simulink model "AC_DCj_iaocuo_simple_hysteresis_1V_commutation_softstart_tuned"  (R2024b)
settings: Solver=FixedStepDiscrete  StartTime=0.0  StopTime=1  FixedStep=1e-7  RelTol=1e-3
libraries: spsMosfetLib x6, spsCurrentMeasurementLib x4, spsSeriesRLCBranchLib x4, slpidlib x3, simulink x3, spsVoltageMeasurementLib x2, spsACVoltageSourceLib x1, dspstat3 x1, sps_lib x1
settings Model: Creator=YuJian  LastModifiedBy=YuJian
settings DataIOCC: ReturnWorkspaceOutputs=off

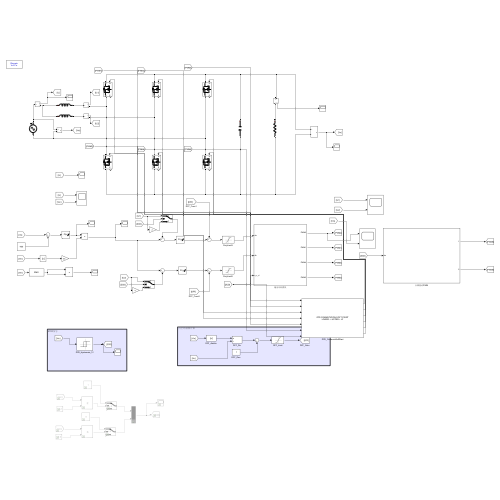
[thumbnail: Simulink's stored preview of the top-level diagram]
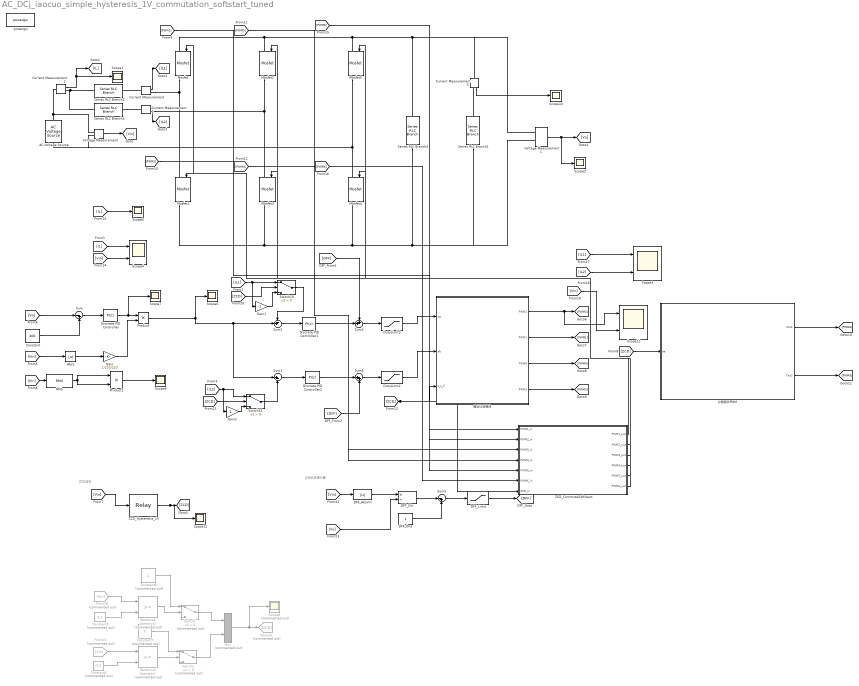
== system AC_DCj_iaocuo_simple_hysteresis_1V_commutation_softstart_tuned ==
  note: 占空比前馈计算
  note: ZCD信号
  AC Voltage Source : spsACVoltageSourceLib/AC Voltage Source  Amplitude=311  Phase=0  Frequency=50  SampleTime=0  Measurements=None  BusType=swing  Pref=10e3  Qref=0  Qmin=-inf  Qmax=+inf
  Abs1 : Abs  SaturateOnIntegerOverflow=off
  Constant : Constant  Value=400
  Constant2 : Constant  Commented=on  Value=-0.2
  Constant5 : Constant  Commented=on  Value=0.2
  Constant6 : Constant  Commented=on
  Constant7 : Constant  Commented=on  Value=0
  Current Measurement{,1..3} (4 alike) : spsCurrentMeasurementLib/Current Measurement  PhasorSimulation=off  OutputType=Complex  PSBequivalent=0
  DFF_AbsVin : Abs  SaturateOnIntegerOverflow=off
  DFF_Div : Product  Inputs=*/
  DFF_Limit : Saturate  UpperLimit=1  LowerLimit=0
  DFF_One : Constant
  Discrete PID Controller : slpidlib/PID Controller  Controller=PI  Form=Parallel  TimeDomain=Discrete-time  UseExternalTs=off  SampleTime=-1  IntegratorMethod=Forward Euler  FilterMethod=Forward Euler  ControllerParametersSource=internal  P=4  I=230  UseKiTs=off  D=0  UseExternalDerivativeSource=off  N=100  UseFilter=on  TunerSelectOption=Transfer Function Based (PID Tuner App)  InitialConditionSource=internal  InitialConditionForIntegrator=0  InitialConditionForFilter=0  DifferentiatorICPrevScaledInput=0  ExternalReset=none  TrackingMode=off  Kt=1  LimitOutput=on  SatLimitsSource=internal  UpperSaturationLimit=5500  LowerSaturationLimit=0  LinearizeAsGain=off  AntiWindupMode=clamping  Kb=1  LimitIntegrator=off  UpperIntegratorSaturationLimit=inf  LowerIntegratorSaturationLimit=-inf  POutMin=[]  POutMax=[]  IOutMin=[]  IOutMax=[]  DOutMin=[]  DOutMax=[]  NOutMin=[]  NOutMax=[]  SumOutMin=[]  SumOutMax=[]  SaturationOutMin=[]  SaturationOutMax=[]  PParamMin=[]  PParamMax=[]  IParamMin=[]  IParamMax=[]  DParamMin=[]  DParamMax=[]  NParamMin=[]  NParamMax=[]  KbParamMin=[]  KbParamMax=[]  KtParamMin=[]  KtParamMax=[]  KbOutMin=[]  KbOutMax=[]  KtOutMin=[]  KtOutMax=[]  IntegratorOutMin=[]  IntegratorOutMax=[]  FilterOutMin=[]  FilterOutMax=[]  SumI1OutMin=[]  SumI1OutMax=[]  SumI2OutMin=[]  SumI2OutMax=[]  SumI3OutMin=[]  SumI3OutMax=[]  SumI4OutMin=[]  SumI4OutMax=[]  SumDOutMin=[]  SumDOutMax=[]  DifferentiatorOutMin=[]  DifferentiatorOutMax=[]  FilterDiffOutCoefMin=[]  FilterDiffOutCoefMax=[]  ReciprocalOutMin=[]  ReciprocalOutMax=[]  SumDenOutMin=[]  SumDenOutMax=[]  SumNumOutMin=[]  SumNumOutMax=[]  DivideOutMin=[]  DivideOutMax=[]  UdiffTsProdOutMin=[]  UdiffTsProdOutMax=[]  NTsProdOutMin=[]  NTsProdOutMax=[]  UintegralTsProdOutMin=[]  UintegralTsProdOutMax=[]  UngainTsProdOutMin=[]  UngainTsProdOutMax=[]  ClampingZeroOutDataTypeStr=Inherit: Inherit via back propagation  ClampingZeroOutMin=[]  ClampingZeroOutMax=[]  FilterDenConstantOutDataTypeStr=Inherit: Inherit via back propagation  FilterDenConstantOutMin=[]  FilterDenConstantOutMax=[]  PCopyOutDataTypeStr=Inherit: Inherit via back propagation  PCopyOutMin=[]  PCopyOutMax=[]  NCopyOutDataTypeStr=Inherit: Inherit via back propagation  NCopyOutMin=[]  NCopyOutMax=[]  IntegratorContinuousStateAttributes=''  IntegratorStateMustResolveToSignalObject=off  IntegratorRTWStateStorageClass=Auto  FilterContinuousStateAttributes=''  FilterStateMustResolveToSignalObject=off  FilterRTWStateStorageClass=Auto  ParallelPVariant=InternalParameters  IdealPVariant=Disabled  IVariant=InternalParameters  DVariant=Disabled  IntegratorVariant=Discrete  SatVariant=Enabled  AWVariant=DiscClampingParallel  PCopyVariant=Disabled  TRVariant=Disabled  FdbkBlocksVariant=Forward  IdealPFdbkVariant=Disabled  SatFdbkVariant=Disabled  DerivativeFilterVariant=Disabled  NVariant=Disabled  NCopyVariant=Disabled_SignalSpec  FilterICVariant=Disabled  IntegratorICVariant=InternalICs  ExternalResetVariant=Disabled  TRSumVariant=Passthrough  SumFdbkVariant=Disabled  SumVariant=Sum_PI  TsampFilterVariant=InternalTs  TsampNgainVariant=Passthrough  TsampIntegralVariant=Disabled_SignalSpec  ExternalSaturationOutDataTypeStr=Inherit: Same as second input  DerivativeSourceVariant=Disabled  PreIntVariant=InternalPreInt
      settings: LibrarySourceBlock=simulink/Discrete/Discrete PID Controller
  Discrete PID Controller1 : slpidlib/PID Controller  Controller=PI  Form=Parallel  TimeDomain=Discrete-time  UseExternalTs=off  SampleTime=-1  IntegratorMethod=Forward Euler  FilterMethod=Forward Euler  ControllerParametersSource=internal  P=0.3  I=300  UseKiTs=off  D=0  UseExternalDerivativeSource=off  N=100  UseFilter=on  TunerSelectOption=Transfer Function Based (PID Tuner App)  InitialConditionSource=internal  InitialConditionForIntegrator=0  InitialConditionForFilter=0  DifferentiatorICPrevScaledInput=0  ExternalReset=none  TrackingMode=off  Kt=1  LimitOutput=on  SatLimitsSource=internal  UpperSaturationLimit=0.3  LowerSaturationLimit=-0.3  LinearizeAsGain=off  AntiWindupMode=clamping  Kb=1  LimitIntegrator=off  UpperIntegratorSaturationLimit=inf  LowerIntegratorSaturationLimit=-inf  POutMin=[]  POutMax=[]  IOutMin=[]  IOutMax=[]  DOutMin=[]  DOutMax=[]  NOutMin=[]  NOutMax=[]  SumOutMin=[]  SumOutMax=[]  SaturationOutMin=[]  SaturationOutMax=[]  PParamMin=[]  PParamMax=[]  IParamMin=[]  IParamMax=[]  DParamMin=[]  DParamMax=[]  NParamMin=[]  NParamMax=[]  KbParamMin=[]  KbParamMax=[]  KtParamMin=[]  KtParamMax=[]  KbOutMin=[]  KbOutMax=[]  KtOutMin=[]  KtOutMax=[]  IntegratorOutMin=[]  IntegratorOutMax=[]  FilterOutMin=[]  FilterOutMax=[]  SumI1OutMin=[]  SumI1OutMax=[]  SumI2OutMin=[]  SumI2OutMax=[]  SumI3OutMin=[]  SumI3OutMax=[]  SumI4OutMin=[]  SumI4OutMax=[]  SumDOutMin=[]  SumDOutMax=[]  DifferentiatorOutMin=[]  DifferentiatorOutMax=[]  FilterDiffOutCoefMin=[]  FilterDiffOutCoefMax=[]  ReciprocalOutMin=[]  ReciprocalOutMax=[]  SumDenOutMin=[]  SumDenOutMax=[]  SumNumOutMin=[]  SumNumOutMax=[]  DivideOutMin=[]  DivideOutMax=[]  UdiffTsProdOutMin=[]  UdiffTsProdOutMax=[]  NTsProdOutMin=[]  NTsProdOutMax=[]  UintegralTsProdOutMin=[]  UintegralTsProdOutMax=[]  UngainTsProdOutMin=[]  UngainTsProdOutMax=[]  ClampingZeroOutDataTypeStr=Inherit: Inherit via back propagation  ClampingZeroOutMin=[]  ClampingZeroOutMax=[]  FilterDenConstantOutDataTypeStr=Inherit: Inherit via back propagation  FilterDenConstantOutMin=[]  FilterDenConstantOutMax=[]  PCopyOutDataTypeStr=Inherit: Inherit via back propagation  PCopyOutMin=[]  PCopyOutMax=[]  NCopyOutDataTypeStr=Inherit: Inherit via back propagation  NCopyOutMin=[]  NCopyOutMax=[]  IntegratorContinuousStateAttributes=''  IntegratorStateMustResolveToSignalObject=off  IntegratorRTWStateStorageClass=Auto  FilterContinuousStateAttributes=''  FilterStateMustResolveToSignalObject=off  FilterRTWStateStorageClass=Auto  ParallelPVariant=InternalParameters  IdealPVariant=Disabled  IVariant=InternalParameters  DVariant=Disabled  IntegratorVariant=Discrete  SatVariant=Enabled  AWVariant=DiscClampingParallel  PCopyVariant=Disabled  TRVariant=Disabled  FdbkBlocksVariant=Forward  IdealPFdbkVariant=Disabled  SatFdbkVariant=Disabled  DerivativeFilterVariant=Disabled  NVariant=Disabled  NCopyVariant=Disabled_SignalSpec  FilterICVariant=Disabled  IntegratorICVariant=InternalICs  ExternalResetVariant=Disabled  TRSumVariant=Passthrough  SumFdbkVariant=Disabled  SumVariant=Sum_PI  TsampFilterVariant=InternalTs  TsampNgainVariant=Passthrough  TsampIntegralVariant=Disabled_SignalSpec  ExternalSaturationOutDataTypeStr=Inherit: Same as second input  DerivativeSourceVariant=Disabled  PreIntVariant=InternalPreInt
      settings: LibrarySourceBlock=simulink/Discrete/Discrete PID Controller
  Discrete PID Controller2 : slpidlib/PID Controller  Controller=PI  Form=Parallel  TimeDomain=Discrete-time  UseExternalTs=off  SampleTime=-1  IntegratorMethod=Forward Euler  FilterMethod=Forward Euler  ControllerParametersSource=internal  P=0.3  I=300  UseKiTs=off  D=0  UseExternalDerivativeSource=off  N=100  UseFilter=on  TunerSelectOption=Transfer Function Based (PID Tuner App)  InitialConditionSource=internal  InitialConditionForIntegrator=0  InitialConditionForFilter=0  DifferentiatorICPrevScaledInput=0  ExternalReset=none  TrackingMode=off  Kt=1  LimitOutput=on  SatLimitsSource=internal  UpperSaturationLimit=0.3  LowerSaturationLimit=-0.3  LinearizeAsGain=off  AntiWindupMode=clamping  Kb=1  LimitIntegrator=off  UpperIntegratorSaturationLimit=inf  LowerIntegratorSaturationLimit=-inf  POutMin=[]  POutMax=[]  IOutMin=[]  IOutMax=[]  DOutMin=[]  DOutMax=[]  NOutMin=[]  NOutMax=[]  SumOutMin=[]  SumOutMax=[]  SaturationOutMin=[]  SaturationOutMax=[]  PParamMin=[]  PParamMax=[]  IParamMin=[]  IParamMax=[]  DParamMin=[]  DParamMax=[]  NParamMin=[]  NParamMax=[]  KbParamMin=[]  KbParamMax=[]  KtParamMin=[]  KtParamMax=[]  KbOutMin=[]  KbOutMax=[]  KtOutMin=[]  KtOutMax=[]  IntegratorOutMin=[]  IntegratorOutMax=[]  FilterOutMin=[]  FilterOutMax=[]  SumI1OutMin=[]  SumI1OutMax=[]  SumI2OutMin=[]  SumI2OutMax=[]  SumI3OutMin=[]  SumI3OutMax=[]  SumI4OutMin=[]  SumI4OutMax=[]  SumDOutMin=[]  SumDOutMax=[]  DifferentiatorOutMin=[]  DifferentiatorOutMax=[]  FilterDiffOutCoefMin=[]  FilterDiffOutCoefMax=[]  ReciprocalOutMin=[]  ReciprocalOutMax=[]  SumDenOutMin=[]  SumDenOutMax=[]  SumNumOutMin=[]  SumNumOutMax=[]  DivideOutMin=[]  DivideOutMax=[]  UdiffTsProdOutMin=[]  UdiffTsProdOutMax=[]  NTsProdOutMin=[]  NTsProdOutMax=[]  UintegralTsProdOutMin=[]  UintegralTsProdOutMax=[]  UngainTsProdOutMin=[]  UngainTsProdOutMax=[]  ClampingZeroOutDataTypeStr=Inherit: Inherit via back propagation  ClampingZeroOutMin=[]  ClampingZeroOutMax=[]  FilterDenConstantOutDataTypeStr=Inherit: Inherit via back propagation  FilterDenConstantOutMin=[]  FilterDenConstantOutMax=[]  PCopyOutDataTypeStr=Inherit: Inherit via back propagation  PCopyOutMin=[]  PCopyOutMax=[]  NCopyOutDataTypeStr=Inherit: Inherit via back propagation  NCopyOutMin=[]  NCopyOutMax=[]  IntegratorContinuousStateAttributes=''  IntegratorStateMustResolveToSignalObject=off  IntegratorRTWStateStorageClass=Auto  FilterContinuousStateAttributes=''  FilterStateMustResolveToSignalObject=off  FilterRTWStateStorageClass=Auto  ParallelPVariant=InternalParameters  IdealPVariant=Disabled  IVariant=InternalParameters  DVariant=Disabled  IntegratorVariant=Discrete  SatVariant=Enabled  AWVariant=DiscClampingParallel  PCopyVariant=Disabled  TRVariant=Disabled  FdbkBlocksVariant=Forward  IdealPFdbkVariant=Disabled  SatFdbkVariant=Disabled  DerivativeFilterVariant=Disabled  NVariant=Disabled  NCopyVariant=Disabled_SignalSpec  FilterICVariant=Disabled  IntegratorICVariant=InternalICs  ExternalResetVariant=Disabled  TRSumVariant=Passthrough  SumFdbkVariant=Disabled  SumVariant=Sum_PI  TsampFilterVariant=InternalTs  TsampNgainVariant=Passthrough  TsampIntegralVariant=Disabled_SignalSpec  ExternalSaturationOutDataTypeStr=Inherit: Same as second input  DerivativeSourceVariant=Disabled  PreIntVariant=InternalPreInt
      settings: LibrarySourceBlock=simulink/Discrete/Discrete PID Controller
  DutyLimit2 : Saturate  UpperLimit=1  LowerLimit=0
  DutyLimit3 : Saturate  UpperLimit=1  LowerLimit=0
  From25 : From  Commented=on  GotoTag=Vin
  From26 : From  Commented=on  GotoTag=Vin
  Gain : Gain  Gain=1/220/220
  Gain1 : Gain  Gain=-1
  Gain2 : Gain  Gain=-1
  Goto16 : Goto  Commented=on  GotoTag=ZCD
  Mosfet{,1..5} (6 alike) : spsMosfetLib/Mosfet  Ron=0.1  Lon=0  Rd=0.01  Vfd=0  IC=0  Rs=1e5  Cs=inf  Measurements=on
  Mux : Mux  Commented=on  Inputs=2
  Product : Product
  Product1 : Product
  RMS : dspstat3/RMS  run=off  directionMode=Each column  dimension=1  InputProcessing=Columns as channels (frame based)  reset_popup=None
  Relational Operator1 : RelationalOperator  Commented=on  Operator=<=  OutDataTypeStr=boolean  RndMeth=Simplest  InputSameDT=off
  Relational Operator2 : RelationalOperator  Commented=on  OutDataTypeStr=boolean  RndMeth=Simplest  InputSameDT=off
  Scope{1..2,5..7,9..11} (8 alike) : Scope
  Scope12 : Scope  NumInputPorts=2
  Scope3 : Scope  NumInputPorts=2
  Scope4 : Scope  NumInputPorts=2
  Scope8 : Scope  Commented=on
  Series RLC Branch1 : spsSeriesRLCBranchLib/Series RLC Branch  LConnTagsString=__new0  RConnTagsString=__new0  BranchType=R  Resistance=29.0909  Inductance=1e-3  SetiL0=off  InitialCurrent=0  Capacitance=1e-6  Setx0=off  InitialVoltage=0  Measurements=None
  Series RLC Branch2 : spsSeriesRLCBranchLib/Series RLC Branch  LConnTagsString=__new0  RConnTagsString=__new0  BranchType=L  Resistance=1  Inductance=3.5e-3  SetiL0=off  InitialCurrent=0  Capacitance=1e-6  Setx0=off  InitialVoltage=0  Measurements=None
  Series RLC Branch3 : spsSeriesRLCBranchLib/Series RLC Branch  LConnTagsString=__new0  RConnTagsString=__new0  BranchType=L  Resistance=1  Inductance=3.5e-3  SetiL0=off  InitialCurrent=0  Capacitance=1e-6  Setx0=off  InitialVoltage=0  Measurements=None
  Series RLC Branch4 : spsSeriesRLCBranchLib/Series RLC Branch  LConnTagsString=__new0  RConnTagsString=__new0  BranchType=C  Resistance=1  Inductance=1e-3  SetiL0=off  InitialCurrent=0  Capacitance=2680e-6  Setx0=on  InitialVoltage=300  Measurements=None
  Sum : Sum  Inputs=|-+
  Sum1 : Sum  Inputs=|+-
  Sum2 : Sum  Inputs=-+|
  Sum3 : Sum  Inputs=++|
  Sum4 : Sum  Inputs=|++
  Sum5 : Sum  Inputs=|-+
  Switch1 : Switch  Commented=on  Criteria=u2 > Threshold  SaturateOnIntegerOverflow=off  InputSameDT=off
  Switch10 : Switch  Criteria=u2 > Threshold  SaturateOnIntegerOverflow=off  InputSameDT=off
  Switch11 : Switch  Criteria=u2 > Threshold  SaturateOnIntegerOverflow=off  InputSameDT=off
  Switch2 : Switch  Commented=on  Criteria=u2 > Threshold  SaturateOnIntegerOverflow=off  InputSameDT=off
  Voltage Measurement : spsVoltageMeasurementLib/Voltage Measurement  PhasorSimulation=off  OutputType=Complex  PSBequivalent=0
  Voltage Measurement1 : spsVoltageMeasurementLib/Voltage Measurement  PhasorSimulation=off  OutputType=Complex  PSBequivalent=0
  ZCD_CommuteSoftStart : Subsystem  Description=|
      | 门极输出统一为0/1。ZCD改变后全部门极关断200ns，然后恢复原PWM。
      | 原来的PWM幅值渐变和100us工频管延迟已经移除。
      | 本模块只处理工频换向，不代替高频桥臂逐周期死区。
      mask Display: disp('ZCD COMMUTATION SOFT START\nLOWER -> UPPER + LF')
  ZCD_Hysteresis_1V : Relay  OnSwitchValue=1  OffSwitchValue=-1  OutDataTypeStr=boolean
  powergui : sps_lib/powergui  Priority=1  SimulationMode=Discrete  SampleTime=1e-7  frequency=60  Iterations=50  frequencyindice=50  Pbase=100e6  ErrMax=1e-4  UnitsV=kV  UnitsW=MW  buscounter=0  FunctionMessages=off  echomessages=off  EnableUseOfTLC=off  CurrentSourceSwitches=off  DisableSnubberDevices=off  DisableRonSwitches=off  DisableVfSwitches=off  DisplayEquations=off  AutomaticDiscreteSolvers=off  SolverType=Tustin/Backward Euler (TBE)  Interpol=off  ExternalGateDelay=off  methode=off  Ts=100  x0status=blocks  SPID=on  SwTol=0  HookPort=off  NonlinearTolerance=1e-4  nMaxIteration=100  ContinueOnMaxIteration=off  RestoreLinks=warning  ResistiveCurrentMeasurement=off  Frange=[0:2:500]  Ylog=off  Xlog=on  ShowGrid=off  save=off  variable=ZData  structure=0  ZoomFFT=off  StartTime=0.0  cycles=1  DisplayStyle=1  fundamental=60  FreqAxis=off  MaxFrequency=1000  frequencyindicesteady=1  RmsSteady=1  display=off
  公频驱动PWM : Subsystem
  输出比较模块 : Subsystem
  wires:
  Current Measurement2/1 -> Scope1/1, [IL]
  Current Measurement/1 -> [IL1]
  Current Measurement1/1 -> [IL2]
  Voltage Measurement1/1 -> Scope2/1, [Vo]
  Voltage Measurement/1 -> [Vin]
  Constant/1 -> Sum/2
  [Vo] -> Sum/1
  Sum/1 -> Discrete PID Controller/1
  Discrete PID Controller/1 -> Scope7/1, Product/1
  Gain/1 -> Product/2
  [Vin] -> RMS/1
  Sum2/1 -> Discrete PID Controller1/1
  Sum1/1 -> Discrete PID Controller2/1
  [IL1] -> Scope3/1
  [IL2] -> Scope3/2
  Product1/1 -> Scope9/1
  Current Measurement3/1 -> Scope10/1
  [Vin] -> Abs1/1
  Abs1/1 -> Gain/1
  [IL1] -> Gain1/1, Switch10/1
  [ZCD] -> Switch10/2
  Gain1/1 -> Switch10/3
  Switch10/1 -> Sum2/1
  [IL2] -> Gain2/1, Switch11/1
  [ZCD] -> Switch11/2
  Gain2/1 -> Switch11/3
  Switch11/1 -> Sum1/2
  DFF_AbsVin/1 -> DFF_Div/1
  Sum5/1 -> DFF_Limit/1
  DFF_Limit/1 -> [DFF]
  [DFF] -> Sum4/2
  Sum4/1 -> DutyLimit2/1
  [Vin] -> DFF_AbsVin/1
  [Vo] -> DFF_Div/2
  Sum3/1 -> DutyLimit3/1
  [DFF] -> Sum3/1
  Discrete PID Controller1/1 -> Sum3/2
  Discrete PID Controller2/1 -> Sum4/1
  输出比较模块/2(PWM1) -> [PWM1]
  输出比较模块/1(PWM2) -> Scope12/1, [PWM2]
  输出比较模块/3(PWM4) -> [PWM4]
  输出比较模块/4(PWM3) -> [PWM3]
  公频驱动PWM/1(Out1) -> [PWM6]
  公频驱动PWM/2(Out2) -> [PWM5]
  [ZCD] -> 公频驱动PWM/1(da)
  [ZCD] -> 输出比较模块/3(z_c_d), ZCD_CommuteSoftStart/7(ZCD_in)
  DFF_One/1 -> Sum5/2
  DFF_Div/1 -> Sum5/1
  [IL] -> Scope4/1
  [Vin] -> Scope4/2
  Product/1 -> Sum1/1, Sum2/2, Scope6/1
  RMS/1 -> Product1/2, Product1/1
  [IL] -> Scope5/1
  From25/1 -> Relational Operator1/1
  Constant2/1 -> Relational Operator1/2
  Relational Operator2/1 -> Switch1/2
  Constant5/1 -> Relational Operator2/2
  From26/1 -> Relational Operator2/1
  Constant6/1 -> Switch1/1
  Relational Operator1/1 -> Switch2/2
  Constant7/1 -> Switch2/1
  Switch1/1 -> Mux/1
  Switch2/1 -> Mux/2
  Mux/1 -> Scope8/1, Goto16/1
  [Vin] -> ZCD_Hysteresis_1V/1
  ZCD_Hysteresis_1V/1 -> [ZCD], Scope11/1
  [Vin] -> Scope12/2
  DutyLimit3/1 -> 输出比较模块/1(da)
  DutyLimit2/1 -> 输出比较模块/2(db)
  [PWM1] -> ZCD_CommuteSoftStart/1(PWM1_in)
  ZCD_CommuteSoftStart/1(PWM1_out) -> Mosfet/1
  [PWM2] -> ZCD_CommuteSoftStart/2(PWM2_in)
  ZCD_CommuteSoftStart/2(PWM2_out) -> Mosfet1/1
  [PWM3] -> ZCD_CommuteSoftStart/3(PWM3_in)
  ZCD_CommuteSoftStart/3(PWM3_out) -> Mosfet2/1
  [PWM4] -> ZCD_CommuteSoftStart/4(PWM4_in)
  ZCD_CommuteSoftStart/4(PWM4_out) -> Mosfet3/1
  [PWM5] -> ZCD_CommuteSoftStart/5(PWM5_in)
  ZCD_CommuteSoftStart/5(PWM5_out) -> Mosfet5/1
  [PWM6] -> ZCD_CommuteSoftStart/6(PWM6_in)
  ZCD_CommuteSoftStart/6(PWM6_out) -> Mosfet4/1
  connections:
  Mosfet/RConn1 -- Current Measurement/RConn1 -- Mosfet1/LConn1
  Mosfet5/RConn1 -- AC Voltage Source/LConn1 -- Voltage Measurement/LConn2 -- Mosfet4/LConn1
  Mosfet/LConn1 -- Mosfet2/LConn1 -- Current Measurement3/LConn1 -- Voltage Measurement1/LConn1 -- Series RLC Branch4/LConn1 -- Mosfet5/LConn1
  Mosfet1/RConn1 -- Voltage Measurement1/LConn2 -- Series RLC Branch1/RConn1 -- Series RLC Branch4/RConn1 -- Mosfet4/RConn1 -- Mosfet3/RConn1
  AC Voltage Source/RConn1 -- Voltage Measurement/LConn1 -- Current Measurement2/LConn1
  Mosfet2/RConn1 -- Current Measurement1/RConn1 -- Mosfet3/LConn1
  Current Measurement/LConn1 -- Series RLC Branch2/RConn1
  Series RLC Branch3/RConn1 -- Current Measurement1/LConn1
  Current Measurement2/RConn1 -- Series RLC Branch2/LConn1 -- Series RLC Branch3/LConn1
  Current Measurement3/RConn1 -- Series RLC Branch1/LConn1

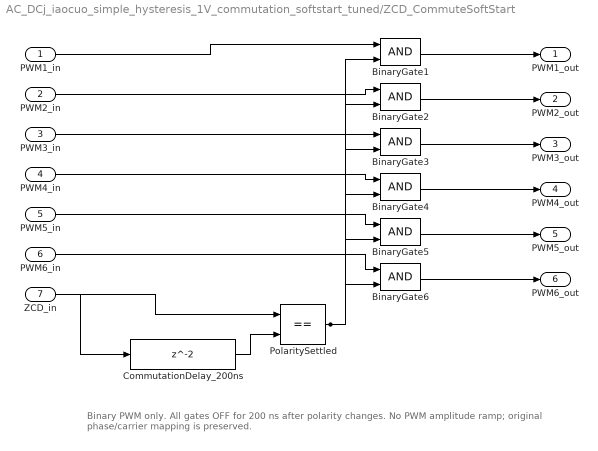
== system AC_DCj_iaocuo_simple_hysteresis_1V_commutation_softstart_tuned/ZCD_CommuteSoftStart ==
  note: Binary PWM only. All gates OFF for 200 ns after polarity changes.\nNo PWM amplitude ramp; original phase/carrier mapping is preserved.
  PWM1_in : Inport
  PWM2_in : Inport  Port=2
  PWM3_in : Inport  Port=3
  PWM4_in : Inport  Port=4
  PWM5_in : Inport  Port=5
  PWM6_in : Inport  Port=6
  ZCD_in : Inport  Port=7
  BinaryGate{1..6} (6 alike) : Logic  AllPortsSameDT=off  OutDataTypeStr=boolean
  CommutationDelay_200ns : Delay  InitialCondition=0  SampleTime=1e-7
  PolaritySettled : RelationalOperator  Operator===  OutDataTypeStr=boolean  RndMeth=Simplest  InputSameDT=off
  PWM1_out : Outport
  PWM2_out : Outport  Port=2
  PWM3_out : Outport  Port=3
  PWM4_out : Outport  Port=4
  PWM5_out : Outport  Port=5
  PWM6_out : Outport  Port=6
  wires:
  ZCD_in/1 -> CommutationDelay_200ns/1, PolaritySettled/1
  CommutationDelay_200ns/1 -> PolaritySettled/2
  PWM1_in/1 -> BinaryGate1/1
  PolaritySettled/1 -> BinaryGate1/2, BinaryGate2/2, BinaryGate3/2, BinaryGate4/2, BinaryGate5/2, BinaryGate6/2
  BinaryGate1/1 -> PWM1_out/1
  PWM2_in/1 -> BinaryGate2/1
  BinaryGate2/1 -> PWM2_out/1
  PWM3_in/1 -> BinaryGate3/1
  BinaryGate3/1 -> PWM3_out/1
  PWM4_in/1 -> BinaryGate4/1
  BinaryGate4/1 -> PWM4_out/1
  PWM5_in/1 -> BinaryGate5/1
  BinaryGate5/1 -> PWM5_out/1
  PWM6_in/1 -> BinaryGate6/1
  BinaryGate6/1 -> PWM6_out/1

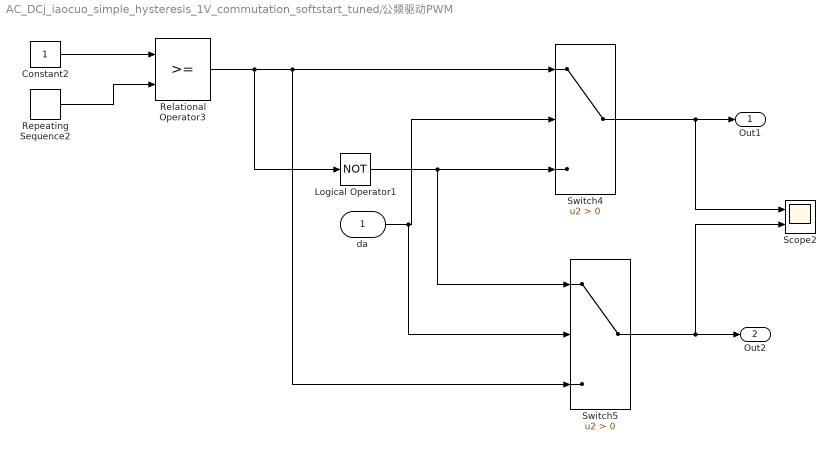
== system AC_DCj_iaocuo_simple_hysteresis_1V_commutation_softstart_tuned/公频驱动PWM ==
  da : Inport
  Constant2 : Constant
  Logical Operator1 : Logic  Operator=NOT  AllPortsSameDT=off  OutDataTypeStr=boolean
  Relational Operator3 : RelationalOperator  OutDataTypeStr=boolean  RndMeth=Simplest  InputSameDT=off
  Repeating Sequence2 : simulink/Sources/Repeating Sequence  rep_seq_t=[0 0.00001 0.00002]  rep_seq_y=[0 1 0]
  Scope2 : Scope  NumInputPorts=2
  Switch4 : Switch  Criteria=u2 > Threshold  SaturateOnIntegerOverflow=off  InputSameDT=off
  Switch5 : Switch  Criteria=u2 > Threshold  SaturateOnIntegerOverflow=off  InputSameDT=off
  Out1 : Outport
  Out2 : Outport  Port=2
  wires:
  Repeating Sequence2/1 -> Relational Operator3/2
  da/1 -> Switch5/2, Switch4/2
  Relational Operator3/1 -> Logical Operator1/1, Switch5/3, Switch4/1
  Switch4/1 -> Scope2/1, Out1/1
  Switch5/1 -> Scope2/2, Out2/1
  Logical Operator1/1 -> Switch5/1, Switch4/3
  Constant2/1 -> Relational Operator3/1

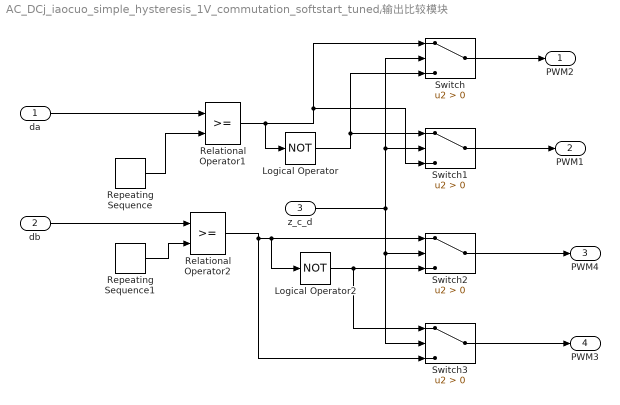
== system AC_DCj_iaocuo_simple_hysteresis_1V_commutation_softstart_tuned/输出比较模块 ==
  da : Inport
  db : Inport  Port=2
  z_c_d : Inport  Port=3
  Logical Operator : Logic  Operator=NOT  AllPortsSameDT=off  OutDataTypeStr=boolean
  Logical Operator2 : Logic  Operator=NOT  AllPortsSameDT=off  OutDataTypeStr=boolean
  Relational Operator1 : RelationalOperator  OutDataTypeStr=boolean  RndMeth=Simplest  InputSameDT=off
  Relational Operator2 : RelationalOperator  OutDataTypeStr=boolean  RndMeth=Simplest  InputSameDT=off
  Repeating Sequence : simulink/Sources/Repeating Sequence  rep_seq_t=[0 0.00001 0.00002]  rep_seq_y=[0 1 0]
  Repeating Sequence1 : simulink/Sources/Repeating Sequence  rep_seq_t=[0 0.00001 0.00002]  rep_seq_y=[1 0 1]
  Switch{,1..3} (4 alike) : Switch  Criteria=u2 > Threshold  SaturateOnIntegerOverflow=off  InputSameDT=off
  PWM2 : Outport
  PWM1 : Outport  Port=2
  PWM4 : Outport  Port=3
  PWM3 : Outport  Port=4
  wires:
  Logical Operator2/1 -> Switch3/1, Switch2/3
  Logical Operator/1 -> Switch1/1, Switch/3
  z_c_d/1 -> Switch3/2, Switch2/2, Switch1/2, Switch/2
  Relational Operator1/1 -> Logical Operator/1, Switch/1, Switch1/3
  Repeating Sequence/1 -> Relational Operator1/2
  Switch2/1 -> PWM4/1
  da/1 -> Relational Operator1/1
  Relational Operator2/1 -> Switch3/3, Logical Operator2/1, Switch2/1
  Repeating Sequence1/1 -> Relational Operator2/2
  Switch3/1 -> PWM3/1
  db/1 -> Relational Operator2/1
  Switch/1 -> PWM2/1
  Switch1/1 -> PWM1/1
